simulink model "pi_pid_control_simulink"  (R2022a)
settings: Solver=VariableStepAuto  StartTime=0.0  StopTime=1200  RelTol=1e-3
undefined symbols (not defined in the file): K_sys, Kp_PI_CHRd, Kp_PI_CHRt, Kp_PI_ZN, Kp_PID_CHRd, Kp_PID_CHRt, Kp_PID_ZN, sigbuilder_block, tau_sys, Td_PI_CHRd, Td_PI_CHRt, Td_PI_ZN, Td_PID_CHRd, Td_PID_CHRt, Td_PID_ZN, theta_sys, Ti_PI_CHRd, Ti_PI_CHRt, Ti_PI_ZN, Ti_PID_CHRd, Ti_PID_CHRt, Ti_PID_ZN
settings Model: Creator=raha  LastModifiedBy=raha

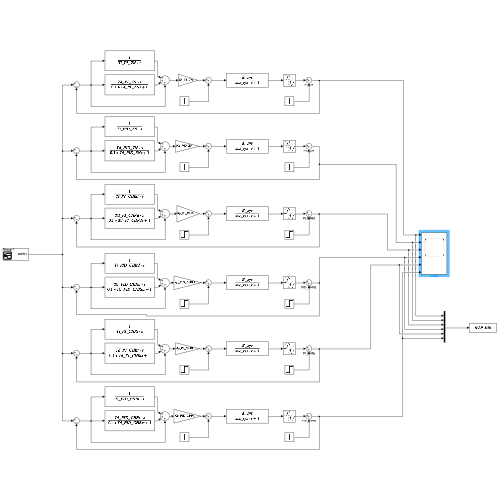
[thumbnail: Simulink's stored preview of the top-level diagram]
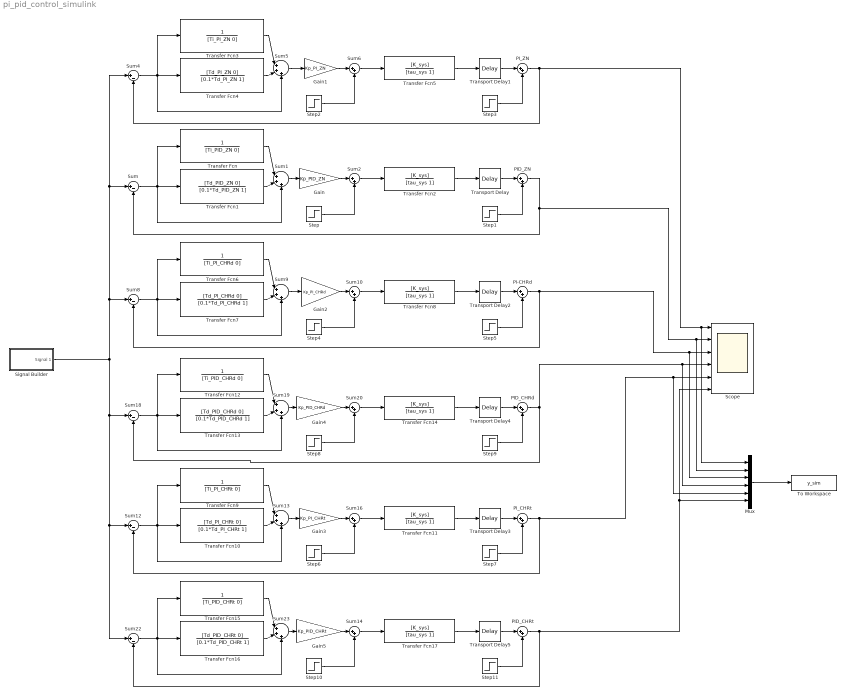
== system pi_pid_control_simulink ==
  Gain : Gain  Gain=Kp_PID_ZN
  Gain1 : Gain  Gain=Kp_PI_ZN
  Gain2 : Gain  Gain=Kp_PI_CHRd
  Gain3 : Gain  Gain=Kp_PI_CHRt
  Gain4 : Gain  Gain=Kp_PID_CHRd
  Gain5 : Gain  Gain=Kp_PID_CHRt
  Mux : Mux  Inputs=6
  PI-CHRd : Sum  Inputs=|++
  PID_CHRd : Sum  Inputs=|++
  PID_CHRt : Sum  Inputs=|++
  PID_ZN : Sum  Inputs=|++
  PI_CHRt : Sum  Inputs=|++
  PI_ZN : Sum  Inputs=|++
  Scope : Scope  NumInputPorts=6
  Signal Builder : Subsystem  Tag=STV Subsys  LoadFcn=sigbuilder_block('load');  StartFcn=sigbuilder_block('start');  StopFcn=sigbuilder_block('stop');  ClipboardFcn=sigbuilder_block('clipboard');  mask(Sigbuilder block){tuvar=[0:10]}
      mask help: Simulink:masks:SigbuilderBlock_MD
      mask init:
      | if ~strcmp(get_param(bdroot(gcbh),'SimulationStatus'),'stopped') tuvar = sigbuilder_block('maskInit'); end
      settings: CopyFcn=sigbuilder_block('copy');  DeleteFcn=sigbuilder_block('delete');  ModelCloseFcn=sigbuilder_block('modelClose');  PreSaveFcn=sigbuilder_block('preSave');  PauseFcn=sigbuilder_block('pause');  ContinueFcn=sigbuilder_block('continue');  NameChangeFcn=sigbuilder_block('namechange');  OpenFcn=sigbuilder_block('open',[367 231 550 400 ]);  CloseFcn=sigbuilder_block('close');
      mask Display: plot(0, 0, 100, 100,[2, 2, 32, 32, 2], [68, 8, 8, 68, 68],[32, 2], [38, 38], [32, 19, 2],[53, 60, 44], [32, 17, 17, 2],[16, 16, 31, 31]);txt = getActiveGroup(gcbh);text(2, 100, txt,'verticalAlignment', 'top');
  Step{,2,4,6,8,10} (6 alike) : Step  Time=600  After=10  SampleTime=0
  Step{1,3,5,7,9,11} (6 alike) : Step  Time=1000  After=10  SampleTime=0
  Sum{,4,8,12,18,22} (6 alike) : Sum  Inputs=|+-
  Sum{1,5,9,13,19,23} (6 alike) : Sum  Inputs=|+++
  Sum{2,6,10,14,16,20} (6 alike) : Sum  Inputs=|++
  To Workspace : ToWorkspace  VariableName=y_sim  SaveFormat=Timeseries  SampleTime=-1
  Transfer Fcn : TransferFcn  Denominator=[Ti_PID_ZN 0]
  Transfer Fcn1 : TransferFcn  Numerator=[Td_PID_ZN 0]  Denominator=[0.1*Td_PID_ZN 1]
  Transfer Fcn10 : TransferFcn  Numerator=[Td_PI_CHRt 0]  Denominator=[0.1*Td_PI_CHRt 1]
  Transfer Fcn{2,5,8,11,14,17} (6 alike) : TransferFcn  Numerator=[K_sys]  Denominator=[tau_sys 1]
  Transfer Fcn12 : TransferFcn  Denominator=[Ti_PID_CHRd 0]
  Transfer Fcn13 : TransferFcn  Numerator=[Td_PID_CHRd 0]  Denominator=[0.1*Td_PID_CHRd 1]
  Transfer Fcn15 : TransferFcn  Denominator=[Ti_PID_CHRt 0]
  Transfer Fcn16 : TransferFcn  Numerator=[Td_PID_CHRt 0]  Denominator=[0.1*Td_PID_CHRt 1]
  Transfer Fcn3 : TransferFcn  Denominator=[Ti_PI_ZN 0]
  Transfer Fcn4 : TransferFcn  Numerator=[Td_PI_ZN 0]  Denominator=[0.1*Td_PI_ZN 1]
  Transfer Fcn6 : TransferFcn  Denominator=[Ti_PI_CHRd 0]
  Transfer Fcn7 : TransferFcn  Numerator=[Td_PI_CHRd 0]  Denominator=[0.1*Td_PI_CHRd 1]
  Transfer Fcn9 : TransferFcn  Denominator=[Ti_PI_CHRt 0]
  Transport Delay{,1..5} (6 alike) : TransportDelay  DelayTime=theta_sys
  wires:
  Sum/1 -> Sum1/3, Transfer Fcn1/1, Transfer Fcn/1
  Transfer Fcn1/1 -> Sum1/2
  Transfer Fcn/1 -> Sum1/1
  Sum1/1 -> Gain/1
  Gain/1 -> Sum2/1
  Sum2/1 -> Transfer Fcn2/1
  Transfer Fcn2/1 -> Transport Delay/1
  Transport Delay/1 -> PID_ZN/1
  Step/1 -> Sum2/2
  Step1/1 -> PID_ZN/2
  PID_ZN/1 -> Mux/2, Scope/2, Sum/2
  PI_ZN/1 -> Mux/1, Scope/1, Sum4/2
  Transfer Fcn4/1 -> Sum5/2
  Transfer Fcn3/1 -> Sum5/1
  Sum5/1 -> Gain1/1
  Step3/1 -> PI_ZN/2
  Transport Delay1/1 -> PI_ZN/1
  Sum4/1 -> Sum5/3, Transfer Fcn4/1, Transfer Fcn3/1
  Gain1/1 -> Sum6/1
  Sum6/1 -> Transfer Fcn5/1
  Transfer Fcn5/1 -> Transport Delay1/1
  Step2/1 -> Sum6/2
  PI-CHRd/1 -> Sum8/2, Mux/3, Scope/3
  Transfer Fcn7/1 -> Sum9/2
  Transfer Fcn6/1 -> Sum9/1
  Sum9/1 -> Gain2/1
  Step5/1 -> PI-CHRd/2
  Transport Delay2/1 -> PI-CHRd/1
  Sum8/1 -> Sum9/3, Transfer Fcn7/1, Transfer Fcn6/1
  Gain2/1 -> Sum10/1
  Sum10/1 -> Transfer Fcn8/1
  Transfer Fcn8/1 -> Transport Delay2/1
  Step4/1 -> Sum10/2
  Signal Builder/1(Signal 1) -> Sum4/1, Sum/1, Sum8/1, Sum22/1, Sum12/1, Sum18/1
  Transfer Fcn16/1 -> Sum23/2
  Transfer Fcn9/1 -> Sum13/1
  Step9/1 -> PID_CHRd/2
  Sum13/1 -> Gain3/1
  Step11/1 -> PID_CHRt/2
  Sum23/1 -> Gain5/1
  Transport Delay5/1 -> PID_CHRt/1
  PID_CHRd/1 -> Mux/4, Scope/4, Sum18/2
  Sum20/1 -> Transfer Fcn14/1
  PI_CHRt/1 -> Mux/5, Scope/5, Sum12/2
  Gain4/1 -> Sum20/1
  Step8/1 -> Sum20/2
  Transfer Fcn13/1 -> Sum19/2
  Transport Delay4/1 -> PID_CHRd/1
  Sum16/1 -> Transfer Fcn11/1
  PID_CHRt/1 -> Mux/6, Scope/6, Sum22/2
  Sum19/1 -> Gain4/1
  Gain5/1 -> Sum14/1
  Transfer Fcn12/1 -> Sum19/1
  Sum18/1 -> Sum19/3, Transfer Fcn13/1, Transfer Fcn12/1
  Transfer Fcn15/1 -> Sum23/1
  Sum22/1 -> Sum23/3, Transfer Fcn16/1, Transfer Fcn15/1
  Transfer Fcn14/1 -> Transport Delay4/1
  Transport Delay3/1 -> PI_CHRt/1
  Gain3/1 -> Sum16/1
  Step7/1 -> PI_CHRt/2
  Transfer Fcn11/1 -> Transport Delay3/1
  Step6/1 -> Sum16/2
  Transfer Fcn10/1 -> Sum13/2
  Sum12/1 -> Sum13/3, Transfer Fcn10/1, Transfer Fcn9/1
  Transfer Fcn17/1 -> Transport Delay5/1
  Step10/1 -> Sum14/2
  Sum14/1 -> Transfer Fcn17/1
  Mux/1 -> To Workspace/1

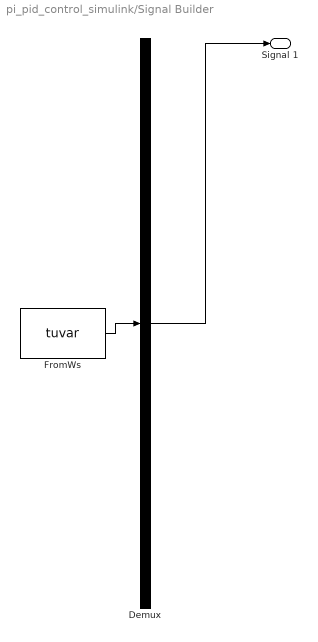
== system pi_pid_control_simulink/Signal Builder ==
  Demux : Demux  Tag=STV Demux  Outputs=1
      settings: DisplayOption=none
  FromWs : FromWorkspace  Tag=STV FromWs  VariableName=tuvar
      SigBuilderData=|
      | common.afterFinalStr = 'Extrapolate'
      | common.sampleTime = 0
      | dataSet.timeRange = [0 1200]
      | dataSet.name = 'Group 1'
      | sbobj.Groups.Name = 'Group 1'
      | sbobj.Groups.Signals.Name = 'Signal 1'
      | sbobj.Groups.Signals.XData = [0 400 400 800 800 1200]
      | sbobj.Groups.Signals.YData = [35 35 55 55 45 45]
      | sbobj.Groups.TimeRange = [0 1200]
  Signal 1 : Outport  Tag=STV Outport
  wires:
  Demux/1 -> Signal 1/1
  FromWs/1 -> Demux/1
